simulink model "EV_Bus_Forward"  (R2025a)
settings: Solver=ode23t  StartTime=0.0  StopTime=CaseStopTime  MaxStep=Comp.MaxStep  RelTol=1e-5  AbsTol=1e-7
model workspace (MAT data in the model file):
  CaseStopTime = 300
  Comp.Tau = 0.976257419556
  Comp.Limit = 5886
  Comp.InitialForce = 0
  Comp.Enable = 1
  Comp.MinAdaptSpeed = 0.5
  Comp.MeasurementStart = 0
  Comp.MeasurementEnd = 300
  Comp.FilterTau = 0.260335311882
  Comp.Deadband = 44.7421939835
  Comp.ErrorClip = 3531.6
  Comp.MaxRate = 1356.558192
  Comp.LogSampleTime = 0.01
  Comp.MaxStep = 0.01
  MeasuredForceBias = 1114.3044183
  MeasuredTraction = [0 0.01 0.02 0.03 0.04 0.05 0.06 0.07 0.08 0.09 0.1 0.11 ... (60002 elements, 30001x2)]
  P.Mass = 20000
  P.Gravity = 9.81
  P.MotorCount = 2
  P.MotorPower = 400000
  P.MotorPeakTorque = 2500
  P.RegenPeakTorque = 1500
  P.RegenPower = 250000
  P.MaxRPM = 12000
  P.GearRatio = 21
  P.GearEfficiency = 0.97
  P.WheelRadius = 0.5
  P.Cd = 0.65
  P.FrontalArea = 8
  P.Crr = 0.008
  P.AirPressure = 101325
  P.AirGasConstant = 287.05
  P.MotorLag = 0.05
  P.BrakeLag = 0.25
  P.BrakeDelay = 0.1
  P.MaxBrakeTorque = 60000
  P.MaxPressure = 8
  P.DriverKp = 0.22
  P.DriverKi = 0.035
  P.DriverKaw = 2
  P.RegenFadeSpeed = 2
  P.RollingFadeSpeed = 0.2
  P.InitialSpeed = 0
  SignalNames = {'Environment_DesiredSpeed_kmph'; 'Environment_RoadSlope_pct'; 'Environment_AmbientTemp_degC'; 'Driver_Accelerator_pct'; 'Driver_Brake_pct'; 'Powertrain_Controller_MotorCommandTotal_Nm'; 'Powertrain_Controller_BrakeDemandWheel_Nm'; 'Electric_Drive_ActualMotorTotal_Nm'; 'Electric_Drive_ActualMotorEach_Nm'; 'Electric_Drive_ActualMotorSpeed_rpm'; 'Electric_Drive_MechanicalPower_kW'; 'Final_Drive_WheelDriveTorque_Nm'; 'Final_Drive_MotorSpeed_rpm'; 'Final_Drive_FinalDriveRatio'; 'Vehicle_Dynamics_VehicleSpeed_mps'; 'Vehicle_Dynamics_VehicleSpeed_kmph'; 'Vehicle_Dynamics_Acceleration_mps2'; 'Vehicle_Dynamics_AccelerationForce_N'; 'Vehicle_Dynamics_GradientForce_N'; 'Vehicle_Dynamics_RollingResistanceForce_N'; 'Vehicle_Dynamics_AerodynamicForce_N'; 'Vehicle_Dynamics_WheelTractionForce_N'; 'Vehicle_Dynamics_DriveForce_N'; 'Vehicle_Dynamics_FrictionBrakeForce_N'; 'Vehicle_Dynamics_StandstillReaction_N'; 'Vehicle_Dynamics_Distance_m'; 'Pneumatic_Brake_FrictionBrakeTorque_Nm'; 'Pneumatic_Brake_ChamberPressure_bar'; 'MeasuredTraction_N'; 'GenericLossForce_N'; 'CorrectedTraction_N'; 'ResidualError_N'; 'RawDifference_N'; 'AppliedGenericLoss_N'; 'DebiasedMeasuredTraction_N'; 'StationaryForceBias_N'; 'FilteredError_N'; 'AdaptationRate_Nps'}
  SlopeProfile = [0  0; 85  0; 100  4; 140  4; 155  0; 180  -3; 200  0; 300  0]
  SpeedProfile = [0  0; 5  0; 25  40; 55  40; 70  0; 85  0; 105  60; 140  60; 160  40; 180  40; 200  0; 225  0; 245  50; 260  50; 280  0; 300  0]
  TemperatureProfile = [0  25; 150  30; 300  35]
values from neighbouring files (symbols this model uses):
  Comp = struct('Tau',baseTau,'Limit',min(0.03*P.Mass*P.Gravity,0.25*driveForce),      'InitialForce',0,'Enable',1,'MinAdaptSpeed',opt(options,'MinAdaptSpeed_mps',0.5),      'MeasurementStart',0,'MeasurementEnd',duration)    [run_EV_Bus_case.m]
  P = getVariable(mw,'P')    [run_EV_Bus_case.m]
(part 1 of 2)
settings Model: Creator=Karuna  LastModifiedBy=Karuna
settings DataIOCC: SignalLogging=off  ReturnWorkspaceOutputs=off

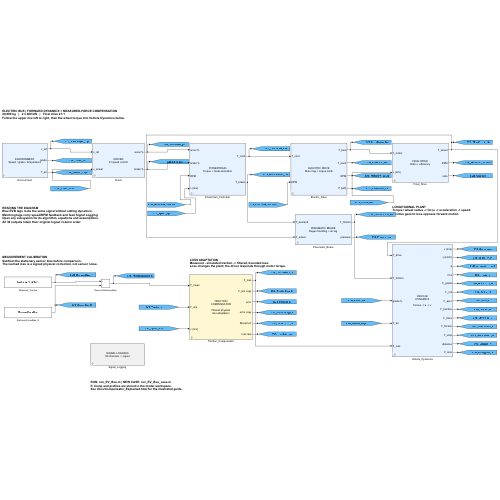
[thumbnail: Simulink's stored preview of the top-level diagram]
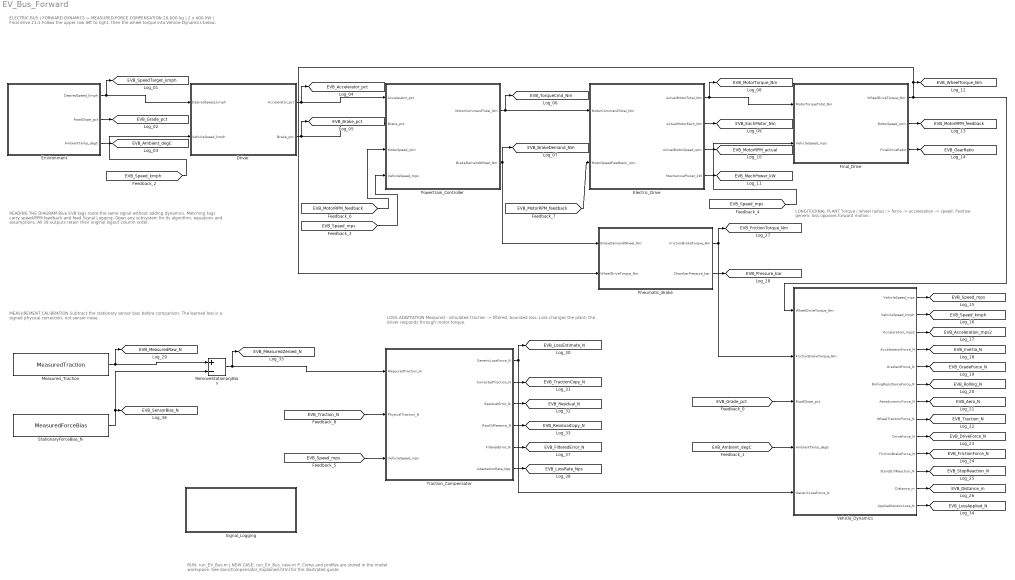
== system EV_Bus_Forward ==
  note: ELECTRIC BUS | FORWARD DYNAMICS + MEASURED-FORCE COMPENSATION
      | 20,000 kg   |   2 x 400 kW   |   Final drive 21:1
      | Follow the upper row left to right, then the wheel torque into Vehicle Dynamics below.
  note: READING THE DIAGRAM
      | Blue EVB tags route the same signal without adding dynamics.
      | Matching tags carry speed/RPM feedback and feed Signal Logging.
      | Open any subsystem for its algorithm, equations and assumptions.
      | All 38 outputs retain their original logout column order.
  note: MEASUREMENT CALIBRATION
      | Subtract the stationary sensor bias before comparison.
      | The learned loss is a signed physical correction, not sensor noise.
  note: LOSS ADAPTATION
      | Measured - simulated traction -> filtered, bounded loss.
      | Loss changes the plant; the driver responds through motor torque.
  note: LONGITUDINAL PLANT
      | Torque / wheel radius -> force -> acceleration -> speed.
      | Positive generic loss opposes forward motion.
  note: RUN: run_EV_Bus.m | NEW CASE: run_EV_Bus_case.m
      | P, Comp and profiles are stored in the model workspace.
      | See docs/Compensator_Explained.html for the illustrated guide.
  Driver : Subsystem  Description=|
      | DRIVER
      | PI control of desired minus actual speed, converted to m/s.
      | Anti-windup and bounded integral state prevent excessive demand.
      | Positive demand: accelerator. Negative demand: brake. Pedals limited to 0..100%.
      | A minimum brake request holds the bus when desired speed is near zero.
      mask help:
      | DRIVER
      | PI control of desired minus actual speed, converted to m/s.
      | Anti-windup and bounded integral state prevent excessive demand.
      | Positive demand: accelerator. Negative demand: brake. Pedals limited to 0..100%.
      | A minimum brake request holds the bus when desired speed is near zero.
      mask Display: disp(sprintf('DRIVER\nPI speed control')); port_label('input',1,'v_ref'); port_label('input',2,'v_actual'); port_label('output',1,'accel %'); port_label('output',2,'brake %');
  Electric_Drive : Subsystem  Description=|
      | ELECTRIC DRIVE
      | First-order torque response with time constant P.MotorLag.
      | Actual torque is clipped to driving/regenerative torque and power envelopes.
      | Identical motors share the combined torque equally.
      | Mechanical power = combined torque * motor angular speed / 1000 (kW).
      mask help:
      | ELECTRIC DRIVE
      | First-order torque response with time constant P.MotorLag.
      | Actual torque is clipped to driving/regenerative torque and power envelopes.
      | Identical motors share the combined torque equally.
      | Mechanical power = combined torque * motor angular speed / 1000 (kW).
      mask Display: disp(sprintf('ELECTRIC DRIVE\nMotor lag + torque limits')); port_label('input',1,'T_cmd'); port_label('input',2,'RPM'); port_label('output',1,'T_total'); port_label('output',2,'T_each'); port_label('output',3,'RPM'); port_label('output',4,'P (kW)');
  Environment : Subsystem  Description=|
      | ENVIRONMENT
      | Desired speed (km/h), grade (%) and ambient temperature (deg C).
      | Profiles are time/value matrices in the model workspace. Grade is positive uphill.
      mask help:
      | ENVIRONMENT
      | Desired speed (km/h), grade (%) and ambient temperature (deg C).
      | Profiles are time/value matrices in the model workspace. Grade is positive uphill.
      mask Display: disp(sprintf('ENVIRONMENT\nSpeed / grade / temperature')); port_label('output',1,'v_ref'); port_label('output',2,'grade'); port_label('output',3,'T_air');
  Final_Drive : Subsystem  Description=|
      | FINAL DRIVE
      | Motor-to-wheel torque conversion with ratio P.GearRatio.
      | Drive: T_wheel = T_motor * ratio * efficiency.
      | Regen: T_wheel = T_motor * ratio / efficiency.
      | Motor RPM = vehicle speed / wheel radius * ratio * 30/pi.
      mask help:
      | FINAL DRIVE
      | Motor-to-wheel torque conversion with ratio P.GearRatio.
      | Drive: T_wheel = T_motor * ratio * efficiency.
      | Regen: T_wheel = T_motor * ratio / efficiency.
      | Motor RPM = vehicle speed / wheel radius * ratio * 30/pi.
      mask Display: disp(sprintf('FINAL DRIVE\nRatio + efficiency')); port_label('input',1,'T_motor'); port_label('input',2,'v (m/s)'); port_label('output',1,'T_wheel'); port_label('output',2,'RPM'); port_label('output',3,'ratio');
  Measured_Traction : FromWorkspace  Description=MeasuredTraction [relative seconds, signed net traction N], configured by run_EV_Bus_case. Supports arbitrary covered duration and timestamp origin. Original timestamps preserved in logout.sourceTime by the runner.  VariableName=MeasuredTraction
  Pneumatic_Brake : Subsystem  Description=|
      | PNEUMATIC SERVICE BRAKE
      | Friction demand = total wheel brake demand minus actual regenerative braking.
      | Clamp demand, convert to pressure, apply air-line delay and chamber filling lag.
      | Pressure is bounded by P.MaxPressure; output torque is positive braking magnitude.
      | This is a reduced-order pressure/torque model, not a valve/reservoir network.
      mask help:
      | PNEUMATIC SERVICE BRAKE
      | Friction demand = total wheel brake demand minus actual regenerative braking.
      | Clamp demand, convert to pressure, apply air-line delay and chamber filling lag.
      | Pressure is bounded by P.MaxPressure; output torque is positive braking magnitude.
      | This is a reduced-order pressure/torque model, not a valve/reservoir network.
      mask Display: disp(sprintf('PNEUMATIC BRAKE\nRegen blending + air lag')); port_label('input',1,'T_demand'); port_label('input',2,'T_wheel'); port_label('output',1,'T_friction'); port_label('output',2,'pressure');
  Powertrain_Controller : Subsystem  Description=|
      | POWERTRAIN CONTROLLER
      | Converts pedals to combined motor torque and total wheel brake demand.
      | Driving torque is positive; regenerative torque is negative.
      | Torque and power limits use P.MotorCount and per-motor ratings.
      | Regeneration fades at low speed; positive drive is inhibited above P.MaxRPM.
      mask help:
      | POWERTRAIN CONTROLLER
      | Converts pedals to combined motor torque and total wheel brake demand.
      | Driving torque is positive; regenerative torque is negative.
      | Torque and power limits use P.MotorCount and per-motor ratings.
      | Regeneration fades at low speed; positive drive is inhibited above P.MaxRPM.
      mask Display: disp(sprintf('POWERTRAIN\nTorque + brake allocation')); port_label('input',1,'accel %'); port_label('input',2,'brake %'); port_label('input',3,'RPM'); port_label('input',4,'v (m/s)'); port_label('output',1,'T_cmd'); port_label('output',2,'T_brake');
  RemoveStationaryBias : Sum  Inputs=+-
  Signal_Logging : Subsystem  Description=|
      | SIGNAL LOGGING
      | Global EVB tags are routing only: no delay, gain or state is introduced.
      | The bus collects all 38 channels in the original column order.
      | To Workspace saves logout as Structure With Time at Comp.LogSampleTime.
      | SignalNames in the model workspace defines the stable column mapping.
      mask help:
      | SIGNAL LOGGING
      | Global EVB tags are routing only: no delay, gain or state is introduced.
      | The bus collects all 38 channels in the original column order.
      | To Workspace saves logout as Structure With Time at Comp.LogSampleTime.
      | SignalNames in the model workspace defines the stable column mapping.
      mask Display: disp(sprintf('SIGNAL LOGGING\n38 channels -> logout'));
  StationaryForceBias_N : Constant  Description=Case-specific measured-force sensor bias. Explicit Bias_N or a user-designated stationary, level, zero-net-traction window; otherwise zero. No universal assumption that the beginning of a recording is stationary.  Value=MeasuredForceBias
  Traction_Compensator : Subsystem  Description=|
      | TRACTION COMPENSATOR - PHYSICAL LOSS ESTIMATOR
      | Error = bias-corrected measured traction minus simulated physical traction.
      | Motion/time gate -> innovation clip -> low-pass filter -> noise deadband.
      | Gate again -> adaptation gain -> rate limit -> bounded integrator -> enable.
      | Positive estimated loss adds resistance; negative loss reduces assumed resistance.
      | Adaptation holds outside valid motion/time intervals. Applied loss fades at rest.
      | The loss changes acceleration and driver demand; traction is NOT replaced by measurement.
      | CorrectedTraction duplicates physical traction; RawDifference is the debiased residual.
      mask help:
      | TRACTION COMPENSATOR - PHYSICAL LOSS ESTIMATOR
      | Error = bias-corrected measured traction minus simulated physical traction.
      | Motion/time gate -> innovation clip -> low-pass filter -> noise deadband.
      | Gate again -> adaptation gain -> rate limit -> bounded integrator -> enable.
      | Positive estimated loss adds resistance; negative loss reduces assumed resistance.
      | Adaptation holds outside valid motion/time intervals. Applied loss fades at rest.
      | The loss changes acceleration and driver demand; traction is NOT replaced by measurement.
      | CorrectedTraction duplicates physical traction; RawDifference is the debiased residual.
      mask Display: disp(sprintf('TRACTION\nCOMPENSATOR\n\nFiltered physical\nloss adaptation')); port_label('input',1,'F_meas'); port_label('input',2,'F_sim'); port_label('input',3,'v (m/s)'); port_label('output',1,'F_loss'); port_label('output',2,'F_sim copy'); port_label('output',3,'error'); port_label('output',4,'error copy'); port_label('output',5,'filtered err'); port_label('output',6,'loss rate');
  Vehicle_Dynamics : Subsystem  Description=|
      | VEHICLE DYNAMICS - FORWARD FORCE BALANCE
      | m*a = F_drive - F_friction - F_grade - F_roll - F_aero - F_loss + F_stop.
      | Integrate acceleration to obtain speed; integrate speed to obtain distance.
      | Reported traction = m*a + F_grade + F_roll + F_aero + F_loss.
      | Grade angle = atan(grade/100); rolling resistance fades near zero speed.
      | Ambient temperature changes air density. Generic loss fades to zero at rest.
      | An ideal standstill reaction prevents reverse motion; no tire-slip or battery model.
      mask help:
      | VEHICLE DYNAMICS - FORWARD FORCE BALANCE
      | m*a = F_drive - F_friction - F_grade - F_roll - F_aero - F_loss + F_stop.
      | Integrate acceleration to obtain speed; integrate speed to obtain distance.
      | Reported traction = m*a + F_grade + F_roll + F_aero + F_loss.
      | Grade angle = atan(grade/100); rolling resistance fades near zero speed.
      | Ambient temperature changes air density. Generic loss fades to zero at rest.
      | An ideal standstill reaction prevents reverse motion; no tire-slip or battery model.
      mask Display: disp(sprintf('VEHICLE\nDYNAMICS\n\nForces -> a -> v')); port_label('input',1,'T_drive'); port_label('input',2,'T_friction'); port_label('input',3,'grade %'); port_label('input',4,'T_air'); port_label('input',5,'F_loss'); port_label('output',1,'v (m/s)'); port_label('output',2,'v (km/h)'); port_label('output',3,'a'); port_label('output',4,'m*a'); port_label('output',5,'F_grade'); port_label('output',6,'F_roll'); port_label('output',7,'F_aero'); port_label('output',8,'F_traction'); port_label('output',9,'F_drive'); port_label('output',10,'F_friction'); port_label('output',11,'F_stop'); port_label('output',12,'distance'); port_label('output',13,'F_loss');
  tag scope: EVB_Acceleration_mps2=global, EVB_Accelerator_pct=global, EVB_Aero_N=global, EVB_Ambient_degC=global, EVB_BrakeDemand_Nm=global, EVB_Brake_pct=global, EVB_Distance_m=global, EVB_DriveForce_N=global, EVB_EachMotor_Nm=global, EVB_FilteredError_N=global, EVB_FrictionForce_N=global, EVB_FrictionTorque_Nm=global, EVB_GearRatio=global, EVB_GradeForce_N=global, EVB_Grade_pct=global, EVB_Inertia_N=global, EVB_LossApplied_N=global, EVB_LossEstimate_N=global, EVB_LossRate_Nps=global, EVB_MeasuredRaw_N=global, EVB_MeasuredZeroed_N=global, EVB_MechPower_kW=global, EVB_MotorRPM_actual=global, EVB_MotorRPM_feedback=global, EVB_MotorTorque_Nm=global, EVB_Pressure_bar=global, EVB_ResidualCopy_N=global, EVB_Residual_N=global, EVB_Rolling_N=global, EVB_SensorBias_N=global, EVB_SpeedTarget_kmph=global, EVB_Speed_kmph=global, EVB_Speed_mps=global, EVB_StopReaction_N=global, EVB_TorqueCmd_Nm=global, EVB_TractionCopy_N=global, EVB_Traction_N=global, EVB_WheelTorque_Nm=global
  wires:
  Traction_Compensator/6(AdaptationRate_Nps) -> [EVB_LossRate_Nps]
  Traction_Compensator/5(FilteredError_N) -> [EVB_FilteredError_N]
  Traction_Compensator/4(RawDifference_N) -> [EVB_ResidualCopy_N]
  Traction_Compensator/3(ResidualError_N) -> [EVB_Residual_N]
  Traction_Compensator/2(CorrectedTraction_N) -> [EVB_TractionCopy_N]
  Pneumatic_Brake/2(ChamberPressure_bar) -> [EVB_Pressure_bar]
  RemoveStationaryBias/1 -> [EVB_MeasuredZeroed_N], Traction_Compensator/1(MeasuredTraction_N)
  Environment/2(RoadSlope_pct) -> [EVB_Grade_pct]
  Environment/3(AmbientTemp_degC) -> [EVB_Ambient_degC]
  Measured_Traction/1 -> [EVB_MeasuredRaw_N], RemoveStationaryBias/1
  StationaryForceBias_N/1 -> [EVB_SensorBias_N], RemoveStationaryBias/2
  Environment/1(DesiredSpeed_kmph) -> [EVB_SpeedTarget_kmph], Driver/1(DesiredSpeed_kmph)
  [EVB_Traction_N] -> Traction_Compensator/2(PhysicalTraction_N)
  [EVB_MotorRPM_feedback] -> Electric_Drive/2(MotorSpeedFeedback_rpm)
  [EVB_MotorRPM_feedback] -> Powertrain_Controller/3(MotorSpeed_rpm)
  [EVB_Speed_mps] -> Traction_Compensator/3(VehicleSpeed_mps)
  [EVB_Speed_mps] -> Final_Drive/2(VehicleSpeed_mps)
  [EVB_Speed_mps] -> Powertrain_Controller/4(VehicleSpeed_mps)
  [EVB_Speed_kmph] -> Driver/2(VehicleSpeed_kmph)
  [EVB_Ambient_degC] -> Vehicle_Dynamics/4(AmbientTemp_degC)
  [EVB_Grade_pct] -> Vehicle_Dynamics/3(RoadSlope_pct)
  Powertrain_Controller/2(BrakeDemandWheel_Nm) -> Pneumatic_Brake/1(BrakeDemandWheel_Nm), [EVB_BrakeDemand_Nm]
  Electric_Drive/1(ActualMotorTotal_Nm) -> Final_Drive/1(MotorTorqueTotal_Nm), [EVB_MotorTorque_Nm]
  Powertrain_Controller/1(MotorCommandTotal_Nm) -> [EVB_TorqueCmd_Nm], Electric_Drive/1(MotorCommandTotal_Nm)
  Final_Drive/2(MotorSpeed_rpm) -> [EVB_MotorRPM_feedback]
  Driver/2(Brake_pct) -> [EVB_Brake_pct], Powertrain_Controller/2(Brake_pct)
  Driver/1(Accelerator_pct) -> Powertrain_Controller/1(Accelerator_pct), [EVB_Accelerator_pct]
  Pneumatic_Brake/1(FrictionBrakeTorque_Nm) -> Vehicle_Dynamics/2(FrictionBrakeTorque_Nm), [EVB_FrictionTorque_Nm]
  Final_Drive/1(WheelDriveTorque_Nm) -> Pneumatic_Brake/2(WheelDriveTorque_Nm), [EVB_WheelTorque_Nm], Vehicle_Dynamics/1(WheelDriveTorque_Nm)
  Vehicle_Dynamics/2(VehicleSpeed_kmph) -> [EVB_Speed_kmph]
  Vehicle_Dynamics/8(WheelTractionForce_N) -> [EVB_Traction_N]
  Traction_Compensator/1(GenericLossForce_N) -> Vehicle_Dynamics/5(GenericLossForce_N), [EVB_LossEstimate_N]
  Vehicle_Dynamics/1(VehicleSpeed_mps) -> [EVB_Speed_mps]
  Electric_Drive/2(ActualMotorEach_Nm) -> [EVB_EachMotor_Nm]
  Electric_Drive/3(ActualMotorSpeed_rpm) -> [EVB_MotorRPM_actual]
  Electric_Drive/4(MechanicalPower_kW) -> [EVB_MechPower_kW]
  Final_Drive/3(FinalDriveRatio) -> [EVB_GearRatio]
  Vehicle_Dynamics/3(Acceleration_mps2) -> [EVB_Acceleration_mps2]
  Vehicle_Dynamics/4(AccelerationForce_N) -> [EVB_Inertia_N]
  Vehicle_Dynamics/5(GradientForce_N) -> [EVB_GradeForce_N]
  Vehicle_Dynamics/6(RollingResistanceForce_N) -> [EVB_Rolling_N]
  Vehicle_Dynamics/7(AerodynamicForce_N) -> [EVB_Aero_N]
  Vehicle_Dynamics/9(DriveForce_N) -> [EVB_DriveForce_N]
  Vehicle_Dynamics/10(FrictionBrakeForce_N) -> [EVB_FrictionForce_N]
  Vehicle_Dynamics/11(StandstillReaction_N) -> [EVB_StopReaction_N]
  Vehicle_Dynamics/12(Distance_m) -> [EVB_Distance_m]
  Vehicle_Dynamics/13(AppliedGenericLoss_N) -> [EVB_LossApplied_N]
